simulink model "Circuito_Online_Definitivo"  (R2024b)
settings: Solver=FixedStepAuto  StartTime=0.0  StopTime=60  RelTol=1e-3
model workspace (MAT data in the model file):
  PCA_coeffK = Simulink.Parameter
  PCA_coeffK.Value = [0.031417995941 -0.0136921286523 0.101212984636 0.106176563865 0.0788268242014 -0.0826314602301 0.096815718661 0.100927555615 0.105773936814 0.00647840331643 0.0950185241378 0.0183038808121 ... (6966 elements, 162x43)]
  PCA_coeffK.Complexity = 'real'
  PCA_coeffK.Dimensions = [162 43]
  PCA_coeffK.DataType = 'auto'
  PCA_mu = Simulink.Parameter
  PCA_mu.Value = [0.0561230714509 -0.282261972362 6.94500497276 2.31958575633 8.7597365107 -8.35900443597 17.1187409467 5440.0049078 2.35464218965 4.55157780819 701.708188274 0.88671875 ... (162 elements, 1x162)]
  PCA_mu.Complexity = 'real'
  PCA_mu.Dimensions = [1 162]
  PCA_mu.DataType = 'auto'
  PCA_sigma = Simulink.Parameter
  PCA_sigma.Value = [0.34168385245 0.471736845585 6.86251142603 1.25143636865 6.83836988941 5.25913074711 10.0563900959 5299.20213776 1.23002081301 1.39530906556 587.851063427 0.97569014465 ... (162 elements, 1x162)]
  PCA_sigma.Complexity = 'real'
  PCA_sigma.Dimensions = [1 162]
  PCA_sigma.DataType = 'auto'
  coeffK29 = [0.031417995941 -0.0136921286523 0.101212984636 0.106176563865 0.0788268242014 -0.0826314602301 0.096815718661 0.100927555615 0.105773936814 0.00647840331643 0.0950185241378 0.0183038808121 ... (4698 elements, 162x29)]
  k_optimum = 43
  k_optimum29 = 29
  mu29 = [0.0561230714509 -0.282261972362 6.94500497276 2.31958575633 8.7597365107 -8.35900443597 17.1187409467 5440.0049078 2.35464218965 4.55157780819 701.708188274 0.88671875 ... (162 elements, 1x162)]
  sigma29 = [0.34168385245 0.471736845585 6.86251142603 1.25143636865 6.83836988941 5.25913074711 10.0563900959 5299.20213776 1.23002081301 1.39530906556 587.851063427 0.97569014465 ... (162 elements, 1x162)]
libraries: visionsources x3, androidsensorlib x2, androiduilib x1, androidaudiovideolib x1
(part 1 of 2)
settings Model: Creator=Marco  LastModifiedBy=Paglia
settings OptimizationCC: EnhancedBackFolding=on  PassReuseOutputArgsThreshold=0  MaxStackSize=64  OptimizeBlockOrder=speed  DifferentSizesBufferReuse=on  OptimizationCustomize=off
settings DebuggingCC: ParameterTunabilityLossMsg=error
settings HardwareCC: ProdBitPerLong=64  ProdLargestAtomicInteger=LongLong  ProdLargestAtomicFloat=Double  ProdLongLongMode=on  ProdHWDeviceType=ARM Compatible->ARM Cortex-A (64-bit)  UseEmbeddedCoderFeatures=off  UseSimulinkCoderFeatures=off
settings RTWCC: Description=Embedded Coder  SystemTargetFile=ert.tlc  HardwareBoard=Android Device (64bit)  TLCOptions="-aInlineSetEventsForThisBaseRateFcn=TLC_FALSE -aSuppressMultiTaskScheduler=TLC_FALSE  -aRateBasedStepFcn=0"  TemplateMakefile=ert_default_tmf  RTWVerbose=off  Toolchain=Android SDK/NDK Tools  GPUComputeCapability=3.5
settings CodeAppCC: ForceParamTrailComments=on  OperatorAnnotations=on
settings ERTTargetCC: ERTCustomFileBanners=off  SupportContinuousTime=on  SupportNonInlinedSFcns=on  RemoveResetFunc=off  ModelStepFunctionPrototypeControlCompliant=off  InlinedParameterPlacement=Hierarchical  DynamicArrayContainerType=coder::array

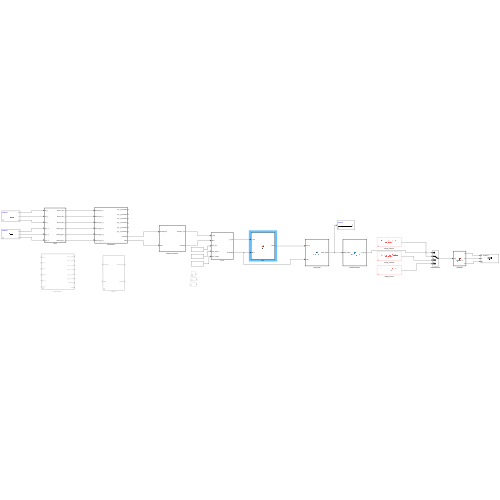
[thumbnail: Simulink's stored preview of the top-level diagram]
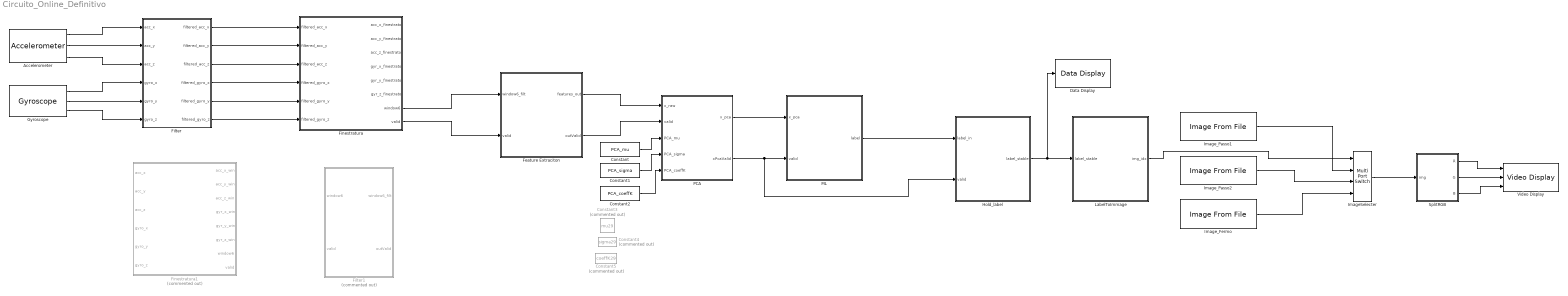
== system Circuito_Online_Definitivo ==
  Accelerometer : androidsensorlib/Accelerometer  OutputVector=off  SampleTime=0.005  BlockPlatform=Android
  Constant : Constant  Value=PCA_mu  VectorParams1D=off
  Constant1 : Constant  Value=PCA_sigma  VectorParams1D=off
  Constant2 : Constant  Value=PCA_coeffK  VectorParams1D=off
  Constant3 : Constant  Commented=on  Value=mu29  VectorParams1D=off
  Constant4 : Constant  Commented=on  Value=sigma29  VectorParams1D=off
  Constant5 : Constant  Commented=on  Value=coeffK29  VectorParams1D=off
  Data Display : androiduilib/Data Display  DataDisplayId=Circuito_Online_Definitivo/Data_Display  Format=Float  Precision=6  SimulateUsing=Code generation  blockPlatform=Android
  Feature Extraciton : MATLAB Function  TreatAsAtomicUnit=on
  Filter : MATLAB Function  TreatAsAtomicUnit=on
  Filter1 : MATLAB Function  Commented=on  TreatAsAtomicUnit=on
  Finestratura : MATLAB Function  TreatAsAtomicUnit=on
  Finestratura1 : MATLAB Function  Commented=on  TreatAsAtomicUnit=on
  Gyroscope : androidsensorlib/Gyroscope  OutputVector=off  SampleTime=0.005  BlockPlatform=Android
  Hold_label : MATLAB Function  TreatAsAtomicUnit=on
  ImageSelecter : MultiPortSwitch  SaturateOnIntegerOverflow=off  InputSameDT=off
  Image_Fermo : visionsources/Image From File  Tag=vipblks_nd  FileName=fermo.png  Ts=0.1  imagePorts=One multidimensional signal  OutPortLabels=R|G|B  ImageDataType=uint8  sdImageDataType=uint(8)  Signed=on  WordLength=16  FractionLengthMode=User-defined  FractionLength=15
  Image_Passo1 : visionsources/Image From File  Tag=vipblks_nd  FileName=passo1.png  Ts=0.1  imagePorts=One multidimensional signal  OutPortLabels=R|G|B  ImageDataType=uint8  sdImageDataType=uint(8)  Signed=on  WordLength=16  FractionLengthMode=User-defined  FractionLength=15
  Image_Passo2 : visionsources/Image From File  Tag=vipblks_nd  FileName=passo2.png  Ts=0.1  imagePorts=One multidimensional signal  OutPortLabels=R|G|B  ImageDataType=uint8  sdImageDataType=uint(8)  Signed=on  WordLength=16  FractionLengthMode=User-defined  FractionLength=15
  LabelToImmage : MATLAB Function  TreatAsAtomicUnit=on
  ML : MATLAB Function  TreatAsAtomicUnit=on
  PCA : MATLAB Function  TreatAsAtomicUnit=on
  SplitRGB : MATLAB Function  TreatAsAtomicUnit=on
  Video Display : androidaudiovideolib/Video Display  BlockPlatform=Android
  wires:
  Filter/2(filtered_acc_y) -> Finestratura/2(filtered_acc_y)
  Filter/4(filtered_gyro_x) -> Finestratura/4(filtered_gyro_x)
  Filter/3(filtered_acc_z) -> Finestratura/3(filtered_acc_z)
  Filter/1(filtered_acc_x) -> Finestratura/1(filtered_acc_x)
  Filter/5(filtered_gyro_y) -> Finestratura/5(filtered_gyro_y)
  Filter/6(filtered_gyro_z) -> Finestratura/6(filtered_gyro_z)
  Feature Extraciton/2(outValid) -> PCA/2(valid)
  Feature Extraciton/1(features_out) -> PCA/1(x_raw)
  PCA/1(x_pca) -> ML/1(x_pca)
  PCA/2(xPcaValid) -> Hold_label/2(valid), ML/2(valid)
  ML/1(label) -> Hold_label/1(label_in)
  Constant/1 -> PCA/3(PCA_mu)
  Constant1/1 -> PCA/4(PCA_sigma)
  Constant2/1 -> PCA/5(PCA_coeffK)
  Hold_label/1(label_stable) -> Data Display/1, LabelToImmage/1(label_stable)
  Image_Passo1/1 -> ImageSelecter/2
  Image_Passo2/1 -> ImageSelecter/3
  Image_Fermo/1 -> ImageSelecter/4
  LabelToImmage/1(img_idx) -> ImageSelecter/1
  SplitRGB/1(R) -> Video Display/1
  SplitRGB/2(G) -> Video Display/2
  SplitRGB/3(B) -> Video Display/3
  ImageSelecter/1 -> SplitRGB/1(img)
  Accelerometer/2 -> Filter/2(acc_y)
  Gyroscope/2 -> Filter/5(gyro_y)
  Accelerometer/1 -> Filter/1(acc_x)
  Accelerometer/3 -> Filter/3(acc_z)
  Gyroscope/1 -> Filter/4(gyro_x)
  Gyroscope/3 -> Filter/6(gyro_z)
  Finestratura/7(window6) -> Feature Extraciton/1(window6_filt)
  Finestratura/8(valid) -> Feature Extraciton/2(valid)
